simulink model "Sinforce"  (R2024a)
settings: Solver=FixedStepAuto  StartTime=0.0  StopTime=20000*Ts  FixedStep=Ts  RelTol=1e-3
undefined symbols (not defined in the file): sys, Ts, U_inf, x0
settings Model: Creator=wolf6845  LastModifiedBy=wolf6845
settings OptimizationCC: DefaultParameterBehavior=Inlined  UseDivisionForNetSlopeComputation=on  GainParamInheritBuiltInType=on  UseFloatMulNetSlope=on  InlineInvariantSignals=on  EfficientFloat2IntCast=on  LifeSpan=1  OptimizeDataStoreBuffers=off  BusAssignmentInplaceUpdate=off
settings DebuggingCC: SFUnexpectedBacktrackingDiag=warning  SFNoUnconditionalDefaultTransitionDiag=warning
settings HardwareCC: ProdLongLongMode=on
settings SFSimCC: MATLABDynamicMemAlloc=off
settings RTWCC: GenerateReport=on  BuildConfiguration=Debug  LaunchReport=on  GPUComputeCapability=3.5
settings CodeAppCC: ForceParamTrailComments=on  EnableCustomComments=on
settings GRTTargetCC: CombineSignalStateStructs=on  MatFileLogging=off  SupportVariableSizeSignals=on  MultiInstanceErrorCode=Warning

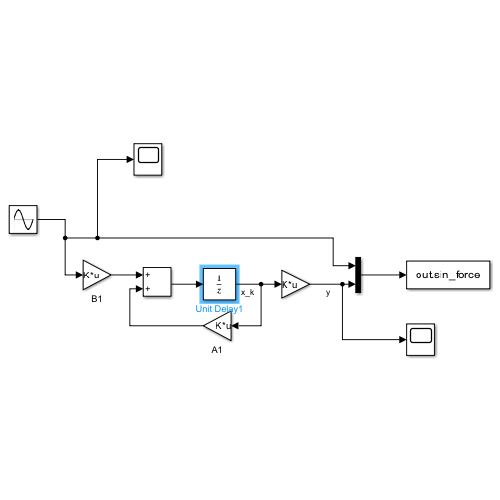
[thumbnail: Simulink's stored preview of the top-level diagram]
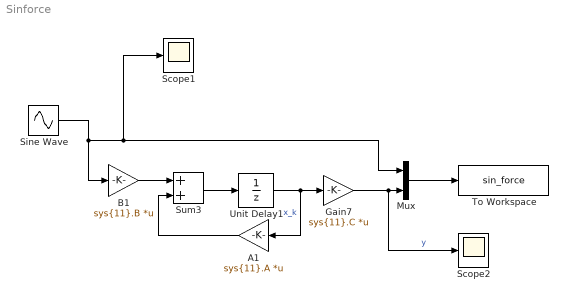
== system Sinforce ==
  A1 : Gain  Gain=sys{11}.A  Multiplication=Matrix(K*u)
  B1 : Gain  Gain=sys{11}.B  Multiplication=Matrix(K*u)
  Gain7 : Gain  Gain=sys{11}.C  Multiplication=Matrix(K*u)
  Mux : Mux  Inputs=2
  Scope1 : Scope
  Scope2 : Scope
  Sine Wave : Sin  Amplitude=U_inf*0.6  Frequency=0.0203  Phase=9*pi/10  SampleTime=0
  Sum3 : Sum
  To Workspace : ToWorkspace  VariableName=sin_force  SampleTime=-1
      settings: Save2DSignal=2-D array (concatenate along first dimension)
  Unit Delay1 : UnitDelay  InitialCondition=x0(1:size(sys{11}.A,1))  SampleTime=Ts  HasFrameUpgradeWarning=on
  wires:
  A1/1 -> Sum3/2
  Sum3/1 -> Unit Delay1/1
  Unit Delay1/1 -> A1/1, Gain7/1  "x_k"
  B1/1 -> Sum3/1
  Mux/1 -> To Workspace/1
  Sine Wave/1 -> B1/1, Scope1/1, Mux/1
  Gain7/1 -> Scope2/1, Mux/2  "y"
